simulink model "Master_Active_Suspension_Simulation"  (R2025b)
settings: Solver=ode45  StartTime=0.0  StopTime=T_stop  MaxStep=1e-3  RelTol=1e-4
PreLoadFcn:
  | parameters;
InitFcn:
  | parameters;
values from neighbouring files (symbols this model uses):
  A = [ 0,                   1,       0,                      -1 ... (first row only)    [plant_model.m]    (also in setup_as.m)
  B = [ 0,         0 ... (first row only)    [plant_model.m]    (also in setup_as.m)
  C = [ 1, 0, 0, 0 ... (first row only)    [plant_model.m]    (also in setup_as.m)
  c1_fixed = 7.00    (= 7)    [parameters.m]
  D = zeros(6, 2)    [plant_model.m]    (also in setup_as.m)
  eps_smc = 0.010    (= 0.01)    [parameters.m]
  F_max = 39.2    [parameters.m]
  k1_fixed = 60.00    (= 60)    [parameters.m]
  k2_fixed = 25.00    (= 25)    [parameters.m]
  K_lqr = lqr_native(A, B(:, 2), Q_lqr, R_lqr)    [parameters.m]
  ROAD_ID = 1    [parameters.m]    (also in run_parameter_sweep.m = r_id; setup_as.m)
undefined symbols (not defined in the file or in its folder): c1_adap, k1_adap, k2_adap
libraries: simulink x6
settings Model: Creator=HP  LastModifiedBy=Santhosh
settings SolverCC: ZeroCrossAlgorithm=Adaptive
settings DebuggingCC: AlgebraicLoopMsg=none
settings RTWCC: GPUComputeCapability=3.5

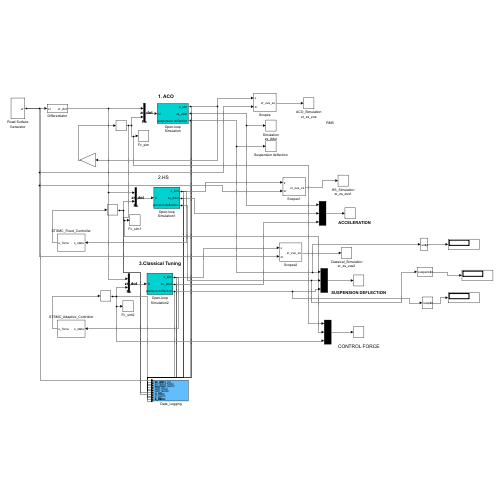
[thumbnail: Simulink's stored preview of the top-level diagram]
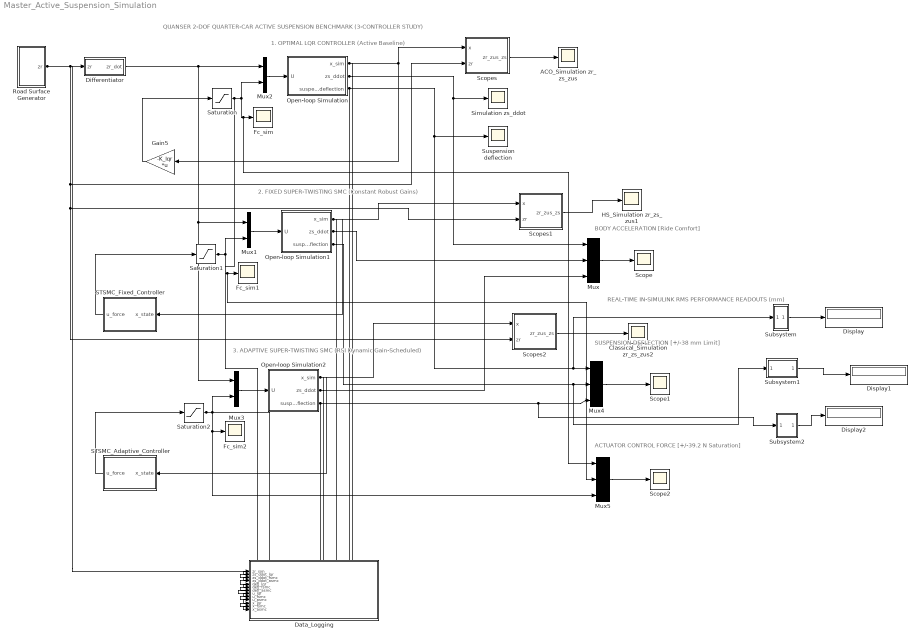
== system Master_Active_Suspension_Simulation ==
  note: REAL-TIME IN-SIMULINK RMS PERFORMANCE READOUTS (mm)
  note: 1. OPTIMAL LQR CONTROLLER (Active Baseline)
  note: SUSPENSION DEFLECTION [+/-38 mm Limit]
  note: ACTUATOR CONTROL FORCE [+/-39.2 N Saturation]
  note: 3. ADAPTIVE SUPER-TWISTING SMC (RSI Dynamic Gain-Scheduled)
  note: 2. FIXED SUPER-TWISTING SMC (Constant Robust Gains)
  note: BODY ACCELERATION [Ride Comfort]
  note: QUANSER 2-DOF QUARTER-CAR ACTIVE SUSPENSION BENCHMARK (3-CONTROLLER STUDY)
  ACO_Simulation zr_zs_zus : Scope
      settings: ActiveDisplayYMinimum=-0.01485  ActiveDisplayYMaximum=0.03485  DataLoggingMaxPoints=300000
  Classical_Simulation zr_zs_zus2 : Scope
      settings: ActiveDisplayYMinimum=-0.01485  ActiveDisplayYMaximum=0.03485  DataLoggingMaxPoints=300000  DataLoggingVariableName=ScopeData6
  Data_Logging : Subsystem
  Differentiator : Subsystem
  Display : Display
  Display1 : Display
  Display2 : Display
  Fc_sim : Scope
      settings: ActiveDisplayYMinimum=-49  ActiveDisplayYMaximum=49  DataLoggingVariableName=ScopeData3
  Fc_sim1 : Scope
      settings: ActiveDisplayYMinimum=-2.01098  ActiveDisplayYMaximum=2.24487  DataLoggingVariableName=ScopeData4
  Fc_sim2 : Scope
      settings: ActiveDisplayYMinimum=-14.56264  ActiveDisplayYMaximum=14.56212  DataLoggingVariableName=ScopeData5
  Gain5 : Gain  Gain=-K_lqr  Multiplication=Matrix(K*u)
  HS_Simulation zr_zs_zus1 : Scope
      settings: ActiveDisplayYMinimum=-0.01485  ActiveDisplayYMaximum=0.03485  DataLoggingMaxPoints=300000  DataLoggingVariableName=ScopeData2
  Mux : Mux  Inputs=3
  Mux1 : Mux  Inputs=2
  Mux2 : Mux  Inputs=2
  Mux3 : Mux  Inputs=2
  Mux4 : Mux  Inputs=3
  Mux5 : Mux  Inputs=3
  Open-loop Simulation : Subsystem
  Open-loop Simulation1 : Subsystem
  Open-loop Simulation2 : Subsystem
  Road Surface Generator : Subsystem
  STSMC_Adaptive_Controller : Subsystem
  STSMC_Fixed_Controller : Subsystem
  Saturation : Saturate  UpperLimit=F_max  LowerLimit=-F_max
  Saturation1 : Saturate  UpperLimit=F_max  LowerLimit=-F_max
  Saturation2 : Saturate  UpperLimit=F_max  LowerLimit=-F_max
  Scope : Scope
      settings: ActiveDisplayYMinimum=-12.27974  ActiveDisplayYMaximum=12.27767  DataLoggingVariableName=ScopeData7
  Scope1 : Scope
      settings: ActiveDisplayYMinimum=-0.04172  ActiveDisplayYMaximum=0.04151  DataLoggingVariableName=ScopeData8
  Scope2 : Scope
      settings: ActiveDisplayYMinimum=-37.18839  ActiveDisplayYMaximum=37.0369  DataLoggingVariableName=ScopeData9
  Scopes : Subsystem
  Scopes1 : Subsystem
  Scopes2 : Subsystem
  Simulation zs_ddot : Scope
      settings: ActiveDisplayYMinimum=-6.91646  ActiveDisplayYMaximum=6.91642  DataLoggingMaxPoints=300000  DataLoggingVariableName=ScopeData10
  Subsystem : Subsystem
  Subsystem1 : Subsystem
  Subsystem2 : Subsystem
  "Suspension deflection " : Scope
      settings: ActiveDisplayYMinimum=-0.03203  ActiveDisplayYMaximum=0.03201  DataLoggingMaxPoints=300000  DataLoggingVariableName=ScopeData11
  wires:
  Mux4/1 -> Scope1/1
  Open-loop Simulation1/3(suspension deflection) -> Subsystem1/1(suspension deflection), Mux4/2, Data_Logging/6(defl_fsmc)
  Saturation1/1 -> Mux1/2, Mux5/2, Fc_sim1/1, Data_Logging/9(u_fsmc)
  Open-loop Simulation/1(x_sim) -> Gain5/1, Scopes/1(x), Data_Logging/11(x_lqr)
  Saturation2/1 -> Mux3/2, Mux5/3, Fc_sim2/1, Data_Logging/10(u_asmc)
  Open-loop Simulation2/3(suspension deflection) -> Subsystem2/1(suspension deflection), Mux4/3, Data_Logging/7(defl_asmc)
  Mux3/1 -> Open-loop Simulation2/1(U)
  Scopes/1(zr_zus_zs) -> ACO_Simulation zr_zs_zus/1
  Road Surface Generator/1(zr) -> Scopes1/2(zr), Scopes2/2(zr), Scopes/2(zr), Differentiator/1(zr), Data_Logging/1(zr_sim)
  Open-loop Simulation2/2(zs_ddot) -> Mux/3, Data_Logging/4(zs_ddot_asmc)
  Open-loop Simulation2/1(x_sim) -> Scopes2/1(x), STSMC_Adaptive_Controller/1(x_state), Data_Logging/13(x_asmc)
  Open-loop Simulation1/2(zs_ddot) -> Mux/2, Data_Logging/3(zs_ddot_fsmc)
  Differentiator/1(zr_dot) -> Mux3/1, Mux1/1, Mux2/1
  Open-loop Simulation/3(suspension deflection) -> Subsystem/1(suspension deflection), Mux4/1, "Suspension deflection "/1, Data_Logging/5(defl_lqr)
  Saturation/1 -> Mux2/2, Mux5/1, Fc_sim/1, Data_Logging/8(u_lqr)
  Open-loop Simulation/2(zs_ddot) -> Mux/1, Simulation zs_ddot/1, Data_Logging/2(zs_ddot_lqr)
  Scopes1/1(zr_zus_zs) -> HS_Simulation zr_zs_zus1/1
  Mux2/1 -> Open-loop Simulation/1(U)
  Mux1/1 -> Open-loop Simulation1/1(U)
  Scopes2/1(zr_zus_zs) -> Classical_Simulation zr_zs_zus2/1
  Open-loop Simulation1/1(x_sim) -> Scopes1/1(x), STSMC_Fixed_Controller/1(x_state), Data_Logging/12(x_fsmc)
  Mux5/1 -> Scope2/1
  Mux/1 -> Scope/1
  Subsystem/1(Out1) -> Display/1
  Subsystem2/1(Out1) -> Display2/1
  Subsystem1/1(Out1) -> Display1/1
  Gain5/1 -> Saturation/1
  STSMC_Fixed_Controller/1(u_force) -> Saturation1/1
  STSMC_Adaptive_Controller/1(u_force) -> Saturation2/1

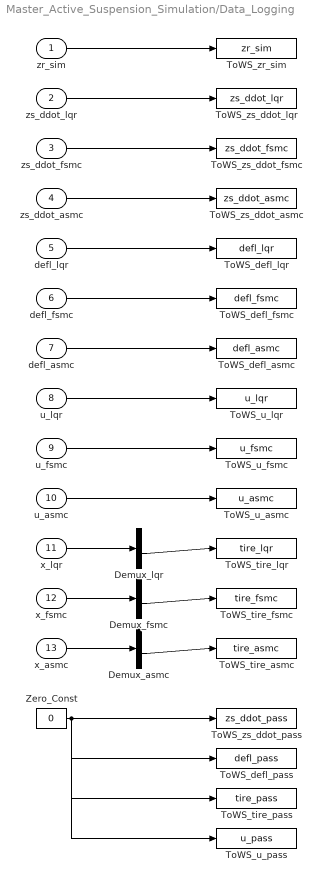
== system Master_Active_Suspension_Simulation/Data_Logging ==
  zr_sim : Inport
  zs_ddot_lqr : Inport  Port=2
  zs_ddot_fsmc : Inport  Port=3
  zs_ddot_asmc : Inport  Port=4
  defl_lqr : Inport  Port=5
  defl_fsmc : Inport  Port=6
  defl_asmc : Inport  Port=7
  u_lqr : Inport  Port=8
  u_fsmc : Inport  Port=9
  u_asmc : Inport  Port=10
  x_lqr : Inport  Port=11
  x_fsmc : Inport  Port=12
  x_asmc : Inport  Port=13
  Demux_asmc : Demux
  Demux_fsmc : Demux
  Demux_lqr : Demux
  ToWS_defl_asmc : ToWorkspace  VariableName=defl_asmc  SampleTime=-1
  ToWS_defl_fsmc : ToWorkspace  VariableName=defl_fsmc  SampleTime=-1
  ToWS_defl_lqr : ToWorkspace  VariableName=defl_lqr  SampleTime=-1
  ToWS_defl_pass : ToWorkspace  VariableName=defl_pass  SampleTime=-1
  ToWS_tire_asmc : ToWorkspace  VariableName=tire_asmc  SampleTime=-1
  ToWS_tire_fsmc : ToWorkspace  VariableName=tire_fsmc  SampleTime=-1
  ToWS_tire_lqr : ToWorkspace  VariableName=tire_lqr  SampleTime=-1
  ToWS_tire_pass : ToWorkspace  VariableName=tire_pass  SampleTime=-1
  ToWS_u_asmc : ToWorkspace  VariableName=u_asmc  SampleTime=-1
  ToWS_u_fsmc : ToWorkspace  VariableName=u_fsmc  SampleTime=-1
  ToWS_u_lqr : ToWorkspace  VariableName=u_lqr  SampleTime=-1
  ToWS_u_pass : ToWorkspace  VariableName=u_pass  SampleTime=-1
  ToWS_zr_sim : ToWorkspace  VariableName=zr_sim  SampleTime=-1
  ToWS_zs_ddot_asmc : ToWorkspace  VariableName=zs_ddot_asmc  SampleTime=-1
  ToWS_zs_ddot_fsmc : ToWorkspace  VariableName=zs_ddot_fsmc  SampleTime=-1
  ToWS_zs_ddot_lqr : ToWorkspace  VariableName=zs_ddot_lqr  SampleTime=-1
  ToWS_zs_ddot_pass : ToWorkspace  VariableName=zs_ddot_pass  SampleTime=-1
  Zero_Const : Constant  Value=0
  wires:
  zr_sim/1 -> ToWS_zr_sim/1
  zs_ddot_lqr/1 -> ToWS_zs_ddot_lqr/1
  zs_ddot_fsmc/1 -> ToWS_zs_ddot_fsmc/1
  zs_ddot_asmc/1 -> ToWS_zs_ddot_asmc/1
  defl_lqr/1 -> ToWS_defl_lqr/1
  defl_fsmc/1 -> ToWS_defl_fsmc/1
  defl_asmc/1 -> ToWS_defl_asmc/1
  u_lqr/1 -> ToWS_u_lqr/1
  u_fsmc/1 -> ToWS_u_fsmc/1
  u_asmc/1 -> ToWS_u_asmc/1
  x_lqr/1 -> Demux_lqr/1
  Demux_lqr/3 -> ToWS_tire_lqr/1
  x_fsmc/1 -> Demux_fsmc/1
  Demux_fsmc/3 -> ToWS_tire_fsmc/1
  x_asmc/1 -> Demux_asmc/1
  Demux_asmc/3 -> ToWS_tire_asmc/1
  Zero_Const/1 -> ToWS_zs_ddot_pass/1, ToWS_defl_pass/1, ToWS_tire_pass/1, ToWS_u_pass/1

== system Master_Active_Suspension_Simulation/Differentiator ==
  zr : Inport
  2nd Order Filter Input ICs3 : Subsystem
  Constant3 : Constant  Value=1000
  Terminator_1 : Terminator
  z4 : Constant
  zr_dot : Outport  VectorParamsAs1DForOutWhenUnconnected=off
  wires:
  Constant3/1 -> 2nd Order Filter Input ICs3/2(Wn)
  z4/1 -> 2nd Order Filter Input ICs3/3(z)
  zr/1 -> 2nd Order Filter Input ICs3/1(In)
  2nd Order Filter Input ICs3/2(Out_dot) -> zr_dot/1
  2nd Order Filter Input ICs3/1(Out) -> Terminator_1/1

== system Master_Active_Suspension_Simulation/Open-loop Simulation ==
  U : Inport
  Demux : Demux  Outputs=[4 2]
  Open-Loop State-Space : StateSpace  A=A  B=B  C=cat(1,eye(4), C)  D=D  InitialCondition=[0;0;0;0]
  Selector : Selector  InputPortWidth=2  IndexOptions=Index vector (dialog)  Indices=[2]  OutputSizes=1
  Selector1 : Selector  InputPortWidth=2  IndexOptions=Index vector (dialog)  Indices=[1]  OutputSizes=1
  x_sim : Outport  VectorParamsAs1DForOutWhenUnconnected=off
  zs_ddot : Outport  Port=2  VectorParamsAs1DForOutWhenUnconnected=off
  suspension deflection : Outport  Port=3  VectorParamsAs1DForOutWhenUnconnected=off
  wires:
  Open-Loop State-Space/1 -> Demux/1
  Demux/1 -> x_sim/1
  U/1 -> Open-Loop State-Space/1
  Demux/2 -> Selector1/1, Selector/1
  Selector/1 -> zs_ddot/1
  Selector1/1 -> suspension deflection/1

== system Master_Active_Suspension_Simulation/Open-loop Simulation1 ==
  U : Inport
  Demux : Demux  Outputs=[4 2]
  Open-Loop State-Space : StateSpace  A=A  B=B  C=cat(1,eye(4), C)  D=D  InitialCondition=[0;0;0;0]
  Selector : Selector  InputPortWidth=2  IndexOptions=Index vector (dialog)  Indices=[2]  OutputSizes=1
  Selector1 : Selector  InputPortWidth=2  IndexOptions=Index vector (dialog)  Indices=[1]  OutputSizes=1
  x_sim : Outport  VectorParamsAs1DForOutWhenUnconnected=off
  zs_ddot : Outport  Port=2  VectorParamsAs1DForOutWhenUnconnected=off
  suspension deflection : Outport  Port=3  VectorParamsAs1DForOutWhenUnconnected=off
  wires:
  Open-Loop State-Space/1 -> Demux/1
  Demux/1 -> x_sim/1
  U/1 -> Open-Loop State-Space/1
  Demux/2 -> Selector1/1, Selector/1
  Selector/1 -> zs_ddot/1
  Selector1/1 -> suspension deflection/1

== system Master_Active_Suspension_Simulation/Open-loop Simulation2 ==
  U : Inport
  Demux : Demux  Outputs=[4 2]
  Open-Loop State-Space : StateSpace  A=A  B=B  C=cat(1,eye(4), C)  D=D  InitialCondition=[0;0;0;0]
  Selector : Selector  InputPortWidth=2  IndexOptions=Index vector (dialog)  Indices=[2]  OutputSizes=1
  Selector1 : Selector  InputPortWidth=2  IndexOptions=Index vector (dialog)  Indices=[1]  OutputSizes=1
  x_sim : Outport  VectorParamsAs1DForOutWhenUnconnected=off
  zs_ddot : Outport  Port=2  VectorParamsAs1DForOutWhenUnconnected=off
  suspension deflection : Outport  Port=3  VectorParamsAs1DForOutWhenUnconnected=off
  wires:
  Open-Loop State-Space/1 -> Demux/1
  Demux/1 -> x_sim/1
  U/1 -> Open-Loop State-Space/1
  Demux/2 -> Selector1/1, Selector/1
  Selector/1 -> zs_ddot/1
  Selector1/1 -> suspension deflection/1

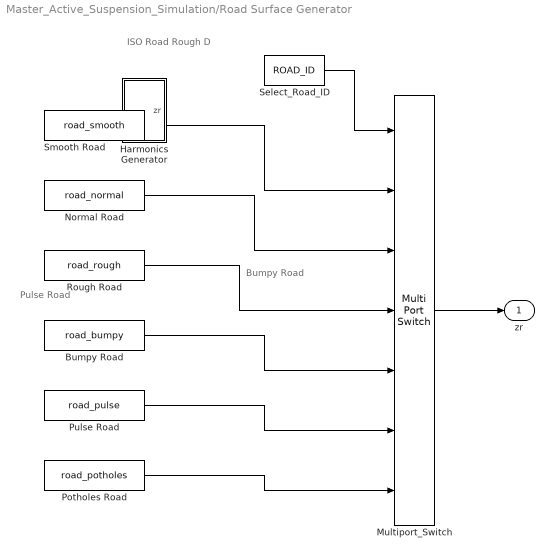
== system Master_Active_Suspension_Simulation/Road Surface Generator ==
  note: Bumpy Road
  note: Pulse Road
  note: ISO Road Rough D
  " Harmonics Generator" : Subsystem
  Bumpy Road : FromWorkspace  VariableName=road_bumpy
  Multiport_Switch : MultiPortSwitch  Inputs=6  SaturateOnIntegerOverflow=off  InputSameDT=off
  Normal Road : FromWorkspace  VariableName=road_normal
  Potholes Road : FromWorkspace  VariableName=road_potholes
  Pulse Road : FromWorkspace  VariableName=road_pulse
  Rough Road : FromWorkspace  VariableName=road_rough
  Select_Road_ID : Constant  Value=ROAD_ID
  Smooth Road : FromWorkspace  VariableName=road_smooth
  zr : Outport  VectorParamsAs1DForOutWhenUnconnected=off
  wires:
  Select_Road_ID/1 -> Multiport_Switch/1
  Smooth Road/1 -> Multiport_Switch/2
  Normal Road/1 -> Multiport_Switch/3
  Rough Road/1 -> Multiport_Switch/4
  Bumpy Road/1 -> Multiport_Switch/5
  Pulse Road/1 -> Multiport_Switch/6
  Potholes Road/1 -> Multiport_Switch/7
  Multiport_Switch/1 -> zr/1

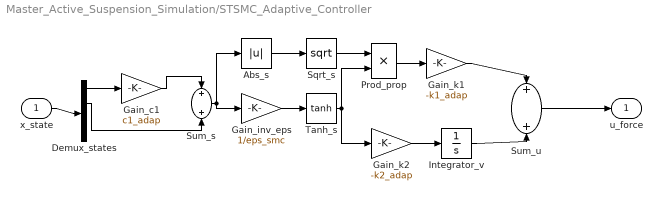
== system Master_Active_Suspension_Simulation/STSMC_Adaptive_Controller ==
  x_state : Inport
  Abs_s : Abs  ZeroCross=off  SaturateOnIntegerOverflow=off
  Demux_states : Demux
  Gain_c1 : Gain  Gain=c1_adap
  Gain_inv_eps : Gain  Gain=1/eps_smc
  Gain_k1 : Gain  Gain=-k1_adap
  Gain_k2 : Gain  Gain=-k2_adap
  Integrator_v : Integrator  LimitOutput=on  UpperSaturationLimit=F_max  LowerSaturationLimit=-F_max
  Prod_prop : Product  Inputs=**
  Sqrt_s : Math  Operator=sqrt
  Sum_s : Sum
  Sum_u : Sum
  Tanh_s : Trigonometry  Operator=tanh
  u_force : Outport
  wires:
  x_state/1 -> Demux_states/1
  Demux_states/1 -> Gain_c1/1
  Gain_c1/1 -> Sum_s/1
  Demux_states/2 -> Sum_s/2
  Sum_s/1 -> Gain_inv_eps/1, Abs_s/1
  Gain_inv_eps/1 -> Tanh_s/1
  Abs_s/1 -> Sqrt_s/1
  Sqrt_s/1 -> Prod_prop/1
  Tanh_s/1 -> Prod_prop/2, Gain_k2/1
  Prod_prop/1 -> Gain_k1/1
  Gain_k2/1 -> Integrator_v/1
  Gain_k1/1 -> Sum_u/1
  Integrator_v/1 -> Sum_u/2
  Sum_u/1 -> u_force/1

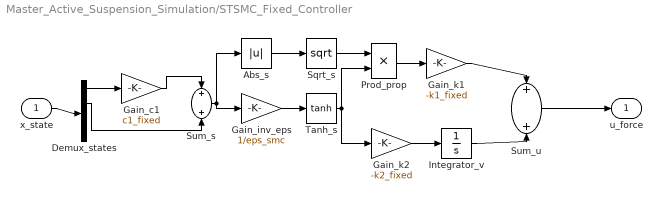
== system Master_Active_Suspension_Simulation/STSMC_Fixed_Controller ==
  x_state : Inport
  Abs_s : Abs  ZeroCross=off  SaturateOnIntegerOverflow=off
  Demux_states : Demux
  Gain_c1 : Gain  Gain=c1_fixed
  Gain_inv_eps : Gain  Gain=1/eps_smc
  Gain_k1 : Gain  Gain=-k1_fixed
  Gain_k2 : Gain  Gain=-k2_fixed
  Integrator_v : Integrator  LimitOutput=on  UpperSaturationLimit=F_max  LowerSaturationLimit=-F_max
  Prod_prop : Product  Inputs=**
  Sqrt_s : Math  Operator=sqrt
  Sum_s : Sum
  Sum_u : Sum
  Tanh_s : Trigonometry  Operator=tanh
  u_force : Outport
  wires:
  x_state/1 -> Demux_states/1
  Demux_states/1 -> Gain_c1/1
  Gain_c1/1 -> Sum_s/1
  Demux_states/2 -> Sum_s/2
  Sum_s/1 -> Gain_inv_eps/1, Abs_s/1
  Gain_inv_eps/1 -> Tanh_s/1
  Abs_s/1 -> Sqrt_s/1
  Sqrt_s/1 -> Prod_prop/1
  Tanh_s/1 -> Prod_prop/2, Gain_k2/1
  Prod_prop/1 -> Gain_k1/1
  Gain_k2/1 -> Integrator_v/1
  Gain_k1/1 -> Sum_u/1
  Integrator_v/1 -> Sum_u/2
  Sum_u/1 -> u_force/1

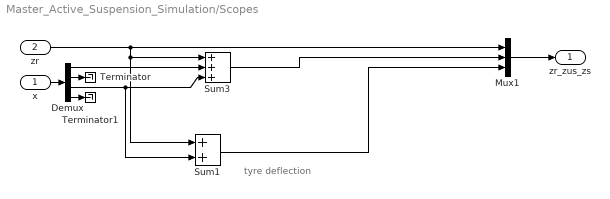
== system Master_Active_Suspension_Simulation/Scopes ==
  note: tyre deflection
  x : Inport
  zr : Inport  Port=2
  Demux : Demux
  Mux1 : Mux  Inputs=3
  Sum1 : Sum  Inputs=2  InputSameDT=on  SaturateOnIntegerOverflow=on  OutDataTypeStr=Inherit: Same as first input
  Sum3 : Sum  Inputs=3  InputSameDT=on  SaturateOnIntegerOverflow=on  OutDataTypeStr=Inherit: Same as first input
  Terminator : Terminator
  Terminator1 : Terminator
  zr_zus_zs : Outport  VectorParamsAs1DForOutWhenUnconnected=off
  wires:
  Demux/1 -> Sum3/2
  Demux/3 -> Sum3/3, Sum1/2
  zr/1 -> Mux1/1, Sum3/1, Sum1/1
  x/1 -> Demux/1
  Mux1/1 -> zr_zus_zs/1
  Demux/2 -> Terminator/1
  Demux/4 -> Terminator1/1
  Sum1/1 -> Mux1/3
  Sum3/1 -> Mux1/2

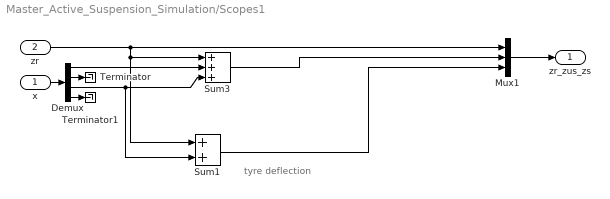
== system Master_Active_Suspension_Simulation/Scopes1 ==
  note: tyre deflection
  x : Inport
  zr : Inport  Port=2
  Demux : Demux
  Mux1 : Mux  Inputs=3
  Sum1 : Sum  Inputs=2  InputSameDT=on  SaturateOnIntegerOverflow=on  OutDataTypeStr=Inherit: Same as first input
  Sum3 : Sum  Inputs=3  InputSameDT=on  SaturateOnIntegerOverflow=on  OutDataTypeStr=Inherit: Same as first input
  Terminator : Terminator
  Terminator1 : Terminator
  zr_zus_zs : Outport  VectorParamsAs1DForOutWhenUnconnected=off
  wires:
  Demux/1 -> Sum3/2
  Demux/3 -> Sum3/3, Sum1/2
  zr/1 -> Mux1/1, Sum3/1, Sum1/1
  x/1 -> Demux/1
  Mux1/1 -> zr_zus_zs/1
  Demux/2 -> Terminator/1
  Demux/4 -> Terminator1/1
  Sum1/1 -> Mux1/3
  Sum3/1 -> Mux1/2

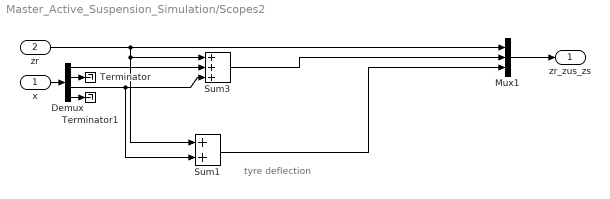
== system Master_Active_Suspension_Simulation/Scopes2 ==
  note: tyre deflection
  x : Inport
  zr : Inport  Port=2
  Demux : Demux
  Mux1 : Mux  Inputs=3
  Sum1 : Sum  Inputs=2  InputSameDT=on  SaturateOnIntegerOverflow=on  OutDataTypeStr=Inherit: Same as first input
  Sum3 : Sum  Inputs=3  InputSameDT=on  SaturateOnIntegerOverflow=on  OutDataTypeStr=Inherit: Same as first input
  Terminator : Terminator
  Terminator1 : Terminator
  zr_zus_zs : Outport  VectorParamsAs1DForOutWhenUnconnected=off
  wires:
  Demux/1 -> Sum3/2
  Demux/3 -> Sum3/3, Sum1/2
  zr/1 -> Mux1/1, Sum3/1, Sum1/1
  x/1 -> Demux/1
  Mux1/1 -> zr_zus_zs/1
  Demux/2 -> Terminator/1
  Demux/4 -> Terminator1/1
  Sum1/1 -> Mux1/3
  Sum3/1 -> Mux1/2

== system Master_Active_Suspension_Simulation/Subsystem ==
  suspension deflection : Inport
  Gain : Gain  Gain=1/10
  Integrator : Integrator  LimitOutput=on  LowerSaturationLimit=0
  Math Function : Math  Operator=square
  Sqrt : Sqrt
  Out1 : Outport
  wires:
  Integrator/1 -> Gain/1
  Math Function/1 -> Integrator/1
  Gain/1 -> Sqrt/1
  Sqrt/1 -> Out1/1
  suspension deflection/1 -> Math Function/1

== system Master_Active_Suspension_Simulation/Subsystem1 ==
  suspension deflection : Inport
  Gain : Gain  Gain=1/10
  Integrator : Integrator  LimitOutput=on  LowerSaturationLimit=0
  Math Function : Math  Operator=square
  Sqrt : Sqrt
  Out1 : Outport
  wires:
  Integrator/1 -> Gain/1
  Math Function/1 -> Integrator/1
  Gain/1 -> Sqrt/1
  Sqrt/1 -> Out1/1
  suspension deflection/1 -> Math Function/1

== system Master_Active_Suspension_Simulation/Subsystem2 ==
  suspension deflection : Inport
  Gain : Gain  Gain=1/10
  Integrator : Integrator  LimitOutput=on  LowerSaturationLimit=0
  Math Function : Math  Operator=square
  Sqrt : Sqrt
  Out1 : Outport
  wires:
  Integrator/1 -> Gain/1
  Math Function/1 -> Integrator/1
  Gain/1 -> Sqrt/1
  Sqrt/1 -> Out1/1
  suspension deflection/1 -> Math Function/1

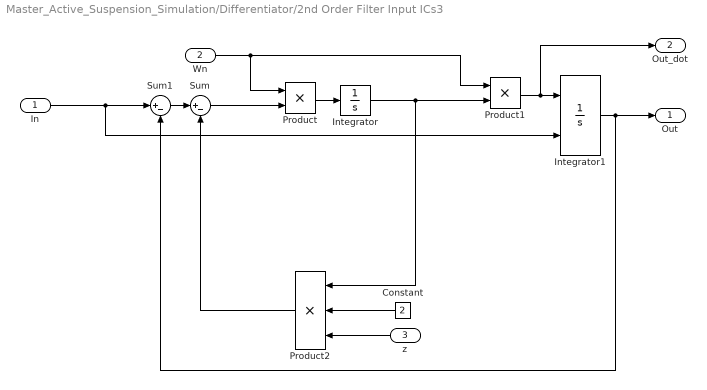
== system Master_Active_Suspension_Simulation/Differentiator/2nd Order Filter Input ICs3 ==
  In : Inport
  Wn : Inport  Port=2
  z : Inport  Port=3
  Constant : Constant  Value=2
  Integrator : Integrator
  Integrator1 : Integrator  InitialConditionSource=external
  Product : Product  RndMeth=Zero
  Product1 : Product  RndMeth=Zero
  Product2 : Product  Inputs=3  RndMeth=Zero
  Sum : Sum  Inputs=|+-
  Sum1 : Sum  Inputs=|+-
  Out : Outport  VectorParamsAs1DForOutWhenUnconnected=off
  Out_dot : Outport  Port=2  VectorParamsAs1DForOutWhenUnconnected=off
  wires:
  Constant/1 -> Product2/2
  z/1 -> Product2/3
  Product2/1 -> Sum/2
  In/1 -> Integrator1/2, Sum1/1
  Sum1/1 -> Sum/1
  Integrator1/1 -> Out/1, Sum1/2
  Integrator/1 -> Product2/1, Product1/2
  Product1/1 -> Out_dot/1, Integrator1/1
  Wn/1 -> Product1/1, Product/1
  Sum/1 -> Product/2
  Product/1 -> Integrator/1

== system Master_Active_Suspension_Simulation/Road Surface Generator/ Harmonics Generator ==
  Constant4 : Constant
  Constant5 : Constant
  Rate Transition : RateTransition
  Repeating Sequence : simulink/Sources/Repeating Sequence  rep_seq_t=[0 30 30.1 ]  rep_seq_y=[1 8 1 ]
  Slider Gain : simulink/Math Operations/Slider Gain  gain=0.0015  low=0  high=0.002
  Slider Gain2 : simulink/Math Operations/Slider Gain  gain=0  low=-10  high=10
  Smooth Parameterized Sin : Subsystem  mask(Smooth Parameterized Sin Wave){}
      mask help:
      | Sin wave that will smoothly and continuously change as input
      | parameters are changed.
      |
      | Out = Amplitude * sin(freq*t) +offset
  Zero-Order Hold : ZeroOrderHold  SampleTime=.1
  zr : Outport  VectorParamsAs1DForOutWhenUnconnected=off
  wires:
  Slider Gain/1 -> Smooth Parameterized Sin/2(Amplitude)
  Slider Gain2/1 -> Smooth Parameterized Sin/3(Offset)
  Constant4/1 -> Slider Gain2/1
  Constant5/1 -> Slider Gain/1
  Repeating Sequence/1 -> Zero-Order Hold/1
  Zero-Order Hold/1 -> Rate Transition/1
  Rate Transition/1 -> Smooth Parameterized Sin/1(freq Hz)
  Smooth Parameterized Sin/1(Sin) -> zr/1

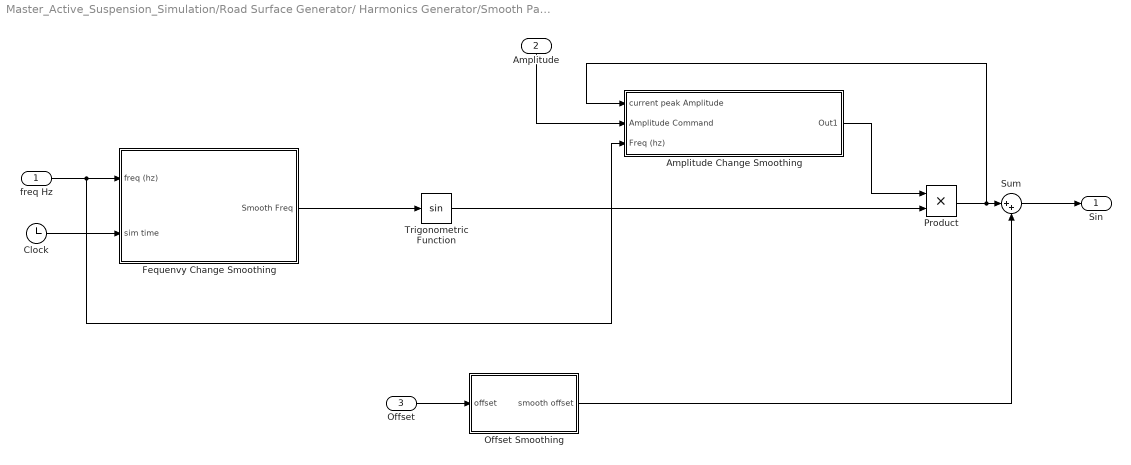
== system Master_Active_Suspension_Simulation/Road Surface Generator/ Harmonics Generator/Smooth Parameterized Sin ==
  freq Hz : Inport
  Amplitude : Inport  Port=2
  Offset : Inport  Port=3
  Amplitude Change Smoothing : Subsystem
  Clock : Clock
  Fequenvy Change Smoothing : Subsystem
  Offset Smoothing : Subsystem
  Product : Product  RndMeth=Zero
  Sum : Sum  Inputs=|++
  Trigonometric Function : Trigonometry
  Sin : Outport  VectorParamsAs1DForOutWhenUnconnected=off
  wires:
  Sum/1 -> Sin/1
  Clock/1 -> Fequenvy Change Smoothing/2(sim time)
  freq Hz/1 -> Fequenvy Change Smoothing/1(freq (hz)), Amplitude Change Smoothing/3(Freq (hz))
  Fequenvy Change Smoothing/1(Smooth Freq) -> Trigonometric Function/1
  Trigonometric Function/1 -> Product/2
  Offset Smoothing/1(smooth offset) -> Sum/2
  Offset/1 -> Offset Smoothing/1(offset)
  Product/1 -> Sum/1, Amplitude Change Smoothing/1(current peak Amplitude)
  Amplitude Change Smoothing/1(Out1) -> Product/1
  Amplitude/1 -> Amplitude Change Smoothing/2(Amplitude Command)

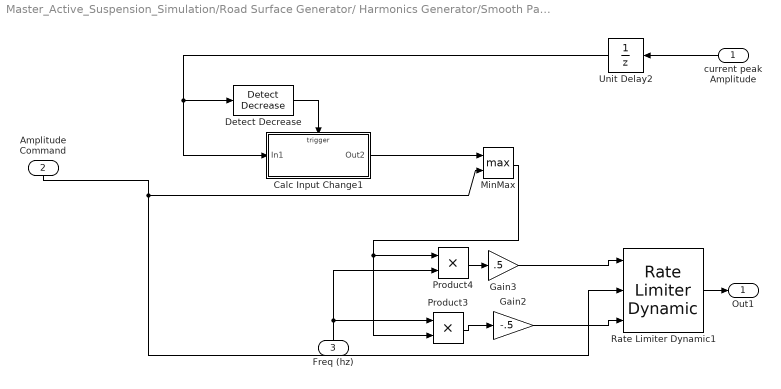
== system Master_Active_Suspension_Simulation/Road Surface Generator/ Harmonics Generator/Smooth Parameterized Sin/Amplitude Change Smoothing ==
  current peak Amplitude : Inport
  Amplitude Command : Inport  Port=2
  Freq (hz) : Inport  Port=3
  Calc Input Change1 : Subsystem  TreatAsAtomicUnit=on
  Detect Decrease : simulink/Logic and Bit Operations/Detect Decrease  vinit=0.0  OutDataTypeStr=uint8
  Gain2 : Gain  Gain=-.5
  Gain3 : Gain  Gain=.5
  MinMax : MinMax  Function=max  Inputs=2
  Product3 : Product  RndMeth=Zero
  Product4 : Product  RndMeth=Zero
  Rate Limiter Dynamic1 : simulink/Discontinuities/Rate Limiter Dynamic
  Unit Delay2 : UnitDelay  SampleTime=-1  HasFrameUpgradeWarning=on
  Out1 : Outport  VectorParamsAs1DForOutWhenUnconnected=off
  wires:
  Gain2/1 -> Rate Limiter Dynamic1/3
  Gain3/1 -> Rate Limiter Dynamic1/1
  Amplitude Command/1 -> MinMax/2, Rate Limiter Dynamic1/2
  Product3/1 -> Gain2/1
  Product4/1 -> Gain3/1
  Detect Decrease/1 -> Calc Input Change1/Trigger
  Calc Input Change1/1(Out2) -> MinMax/1
  Unit Delay2/1 -> Calc Input Change1/1(In1), Detect Decrease/1
  MinMax/1 -> Product4/1, Product3/2
  current peak Amplitude/1 -> Unit Delay2/1
  Freq (hz)/1 -> Product3/1, Product4/2
  Rate Limiter Dynamic1/1 -> Out1/1

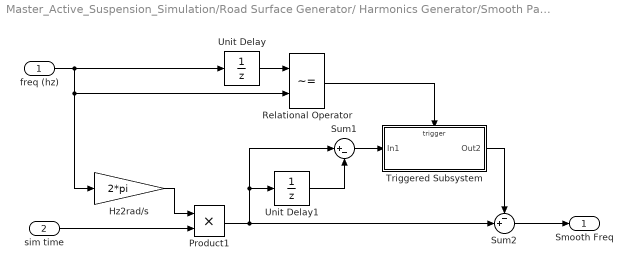
== system Master_Active_Suspension_Simulation/Road Surface Generator/ Harmonics Generator/Smooth Parameterized Sin/Fequenvy Change Smoothing ==
  freq (hz) : Inport
  sim time : Inport  Port=2
  Hz2rad/s : Gain  Gain=2*pi
  Product1 : Product  RndMeth=Zero
  Relational Operator : RelationalOperator  Operator=~=  OutDataTypeStr=boolean  InputSameDT=off
  Sum1 : Sum  Inputs=|+-
  Sum2 : Sum  Inputs=-+|
  Triggered Subsystem : Subsystem  TreatAsAtomicUnit=on
  Unit Delay : UnitDelay  SampleTime=-1  HasFrameUpgradeWarning=on
  Unit Delay1 : UnitDelay  SampleTime=-1  HasFrameUpgradeWarning=on
  Smooth Freq : Outport  VectorParamsAs1DForOutWhenUnconnected=off
  wires:
  Triggered Subsystem/1(Out2) -> Sum2/1
  Unit Delay1/1 -> Sum1/2
  Relational Operator/1 -> Triggered Subsystem/Trigger
  Sum1/1 -> Triggered Subsystem/1(In1)
  Unit Delay/1 -> Relational Operator/1
  Product1/1 -> Sum2/2, Sum1/1, Unit Delay1/1
  freq (hz)/1 -> Unit Delay/1, Relational Operator/2, Hz2rad/s/1
  Sum2/1 -> Smooth Freq/1
  sim time/1 -> Product1/2
  Hz2rad/s/1 -> Product1/1

== system Master_Active_Suspension_Simulation/Road Surface Generator/ Harmonics Generator/Smooth Parameterized Sin/Offset Smoothing ==
  offset : Inport
  Abs : Abs  SaturateOnIntegerOverflow=off
  Abs1 : Abs  SaturateOnIntegerOverflow=off
  Gain : Gain
  Gain1 : Gain  Gain=-1
  MinMax1 : MinMax  Function=max  Inputs=2
  Rate Limiter Dynamic : simulink/Discontinuities/Rate Limiter Dynamic
  Unit Delay3 : UnitDelay  SampleTime=-1  HasFrameUpgradeWarning=on
  smooth offset : Outport  VectorParamsAs1DForOutWhenUnconnected=off
  wires:
  Rate Limiter Dynamic/1 -> Abs1/1, smooth offset/1
  offset/1 -> Rate Limiter Dynamic/2, Abs/1
  Gain1/1 -> Rate Limiter Dynamic/3
  Gain/1 -> Rate Limiter Dynamic/1
  MinMax1/1 -> Unit Delay3/1
  Unit Delay3/1 -> Gain/1, Gain1/1
  Abs/1 -> MinMax1/2
  Abs1/1 -> MinMax1/1

== system Master_Active_Suspension_Simulation/Road Surface Generator/ Harmonics Generator/Smooth Parameterized Sin/Amplitude Change Smoothing/Calc Input Change1 ==
  In1 : Inport
  Trigger : TriggerPort  VariantControl=(inherit)
  Out2 : Outport  InitialOutput=1000  VectorParamsAs1DForOutWhenUnconnected=off
  wires:
  In1/1 -> Out2/1

== system Master_Active_Suspension_Simulation/Road Surface Generator/ Harmonics Generator/Smooth Parameterized Sin/Fequenvy Change Smoothing/Triggered Subsystem ==
  In1 : Inport
  Trigger : TriggerPort  VariantControl=(inherit)
  Sum1 : Sum
  Unit Delay1 : UnitDelay  SampleTime=-1  HasFrameUpgradeWarning=on
  Out2 : Outport  InitialOutput=0  VectorParamsAs1DForOutWhenUnconnected=off
  wires:
  Unit Delay1/1 -> Sum1/1
  Sum1/1 -> Unit Delay1/1, Out2/1
  In1/1 -> Sum1/2
